simulink library "axes_transformation_lib"  (R2018b)
settings: Solver=VariableStepAuto  StartTime=0.0  StopTime=10.0  RelTol=1e-3
settings Model: Creator=Ybeyer  LastModifiedBy=yannic
settings DebuggingCC: LibraryContextMissingDiagnostic=none
settings SFSimCC: SimUseLocalCustomCode=off
settings RTWCC: RTWUseLocalCustomCode=off
settings CodeAppCC: StateflowObjectComments=on

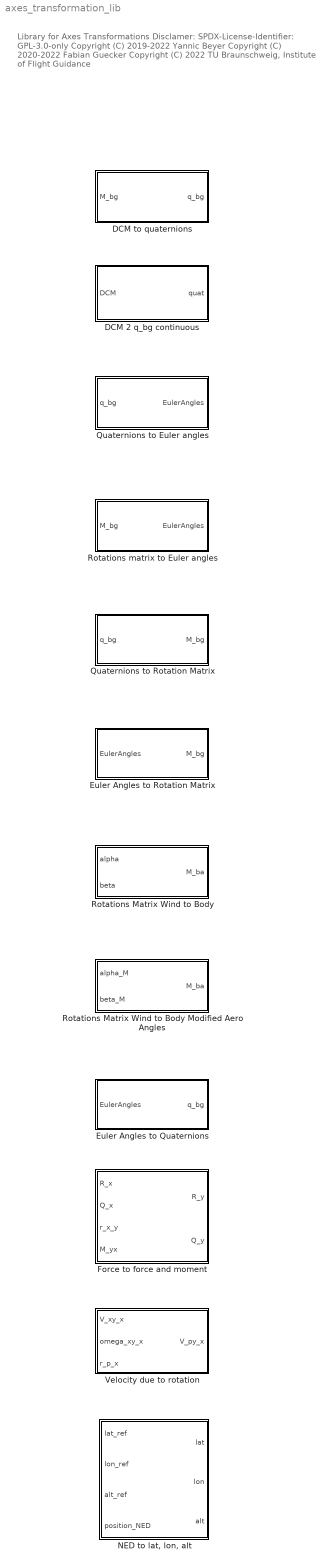
== system axes_transformation_lib ==
  note: Library for Axes Transformations
      |
      | Disclamer:
      | SPDX-License-Identifier: GPL-3.0-only
      |
      | Copyright (C) 2019-2022 Yannic Beyer
      | Copyright (C) 2020-2022 Fabian Guecker
      | Copyright (C) 2022 TU Braunschweig, Institute of Flight Guidance
  DCM 2 q_bg continuous : Subsystem
      mask DialogControl DescGroupVar Prompt: Get quaternions from DCM without discontinuities
      mask DialogControl DescTextVar Prompt: Look inside the block (and function) for more information.
  DCM to quaternions : MATLAB Function  TreatAsAtomicUnit=on
  Euler Angles to Quaternions : MATLAB Function  TreatAsAtomicUnit=on
  Euler Angles to Rotation Matrix : MATLAB Function  TreatAsAtomicUnit=on
  Force to force and moment : MATLAB Function  TreatAsAtomicUnit=on
  "NED to lat, lon, alt" : MATLAB Function  TreatAsAtomicUnit=on
  Quaternions to Euler angles : MATLAB Function  TreatAsAtomicUnit=on
  Quaternions to Rotation Matrix : MATLAB Function  TreatAsAtomicUnit=on
  Rotations Matrix Wind to Body : MATLAB Function  TreatAsAtomicUnit=on
  Rotations Matrix Wind to Body Modified Aero Angles : MATLAB Function  TreatAsAtomicUnit=on
  Rotations matrix to Euler angles : MATLAB Function  TreatAsAtomicUnit=on
  Velocity due to rotation : MATLAB Function  TreatAsAtomicUnit=on

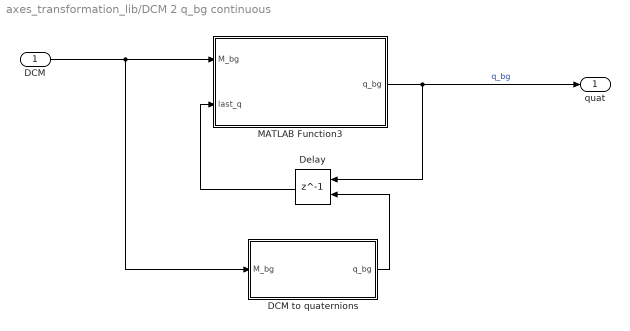
== system axes_transformation_lib/DCM 2 q_bg continuous ==
  DCM : Inport
  DCM to quaternions : MATLAB Function  TreatAsAtomicUnit=on
  Delay : Delay  DelayLength=1  InitialConditionSource=Input port
      settings: InputPortMap=u0,p4
  MATLAB Function3 : MATLAB Function  TreatAsAtomicUnit=on
  quat : Outport
  wires:
  Delay/1 -> MATLAB Function3/2(last_q)
  DCM/1 -> DCM to quaternions/1(M_bg), MATLAB Function3/1(M_bg)
  MATLAB Function3/1(q_bg) -> Delay/1, quat/1  "q_bg"
  DCM to quaternions/1(q_bg) -> Delay/2

== matlab function axes_transformation_lib/Rotations matrix to Euler angles ==
  data: M_bg input; EulerAngles output
function EulerAngles  = fcn( M_bg ) %#codegen
EulerAngles  = dcm2Euler( M_bg );

== matlab function axes_transformation_lib/Quaternions to Euler angles ==
  data: q_bg input; EulerAngles output
function EulerAngles  = fcn( q_bg ) %#codegen
EulerAngles  = quat2Euler( q_bg );

== matlab function axes_transformation_lib/Quaternions to Rotation Matrix ==
  data: q_bg input; M_bg output
function M_bg = fcn(q_bg) %#codegen
M_bg = quat2Dcm(q_bg);

== matlab function axes_transformation_lib/Euler Angles to Rotation Matrix ==
  data: EulerAngles input; M_bg output
function M_bg = fcn(EulerAngles) %#codegen
M_bg = euler2Dcm(EulerAngles);

== matlab function axes_transformation_lib/Rotations Matrix Wind to Body Modified Aero Angles ==
  data: alpha_M input; M_ba output; beta_M input
function M_ba = fcn( alpha_M, beta_M ) %#codegen
M_ba = dcmBaFromAeroAnglesMod( alpha_M, beta_M );

== matlab function axes_transformation_lib/Rotations Matrix Wind to Body ==
  data: alpha input; M_ba output; beta input
function M_ba = fcn( alpha, beta ) %#codegen
M_ba = dcmBaFromAeroAngles( alpha, beta );

== matlab function axes_transformation_lib/Euler Angles to Quaternions ==
  data: EulerAngles input; q_bg output
function q_bg = fcn(EulerAngles) %#codegen
q_bg = euler2Quat(EulerAngles);

== matlab function axes_transformation_lib/Force to force and moment ==
  data: R_x input; Q_x input; r_x_y input; R_y output; M_yx input; Q_y output
function [ R_y, Q_y ] = fcn( R_x, Q_x, r_x_y, M_yx )%#codegen
[ R_y, Q_y ] = forceMomentTransform( R_x, Q_x, r_x_y, M_yx );

== matlab function axes_transformation_lib/Velocity due to rotation ==
  data: V_xy_x input; V_py_x output; omega_xy_x input; r_p_x input
function V_py_x = fcn( V_xy_x, omega_xy_x, r_p_x )%#codegen
V_py_x = velocityFromRot( V_xy_x, omega_xy_x, r_p_x );

== matlab function axes_transformation_lib/DCM 2 q_bg continuous/MATLAB Function3 ==
  data: M_bg input; q_bg output; last_q input
function q_bg  = dcm2QuatCont( M_bg, last_q )
q_bg  = dcm2QuatCont( M_bg, last_q );
end

== matlab function axes_transformation_lib/DCM to quaternions ==
  data: M_bg input; q_bg output
function q_bg  = fcn( M_bg ) %#codegen
q_bg  = dcm2Quat( M_bg );

== matlab function axes_transformation_lib/NED to lat, lon, alt ==
  data: lat_ref input; lat output; lon_ref input; alt_ref input; position_NED input; lon output; alt output
function [lat, lon, alt] = fcn(lat_ref, lon_ref, alt_ref, position_NED) %#codegen
    [lat, lon, alt] = ned2Lla(lat_ref, lon_ref, alt_ref, position_NED);
end

== matlab function axes_transformation_lib/DCM 2 q_bg continuous/DCM to quaternions ==
  data: M_bg input; q_bg output
function q_bg  = fcn( M_bg ) %#codegen
q_bg  = dcm2Quat( M_bg );
